simulink model "sfSelfBroadcastError"  (R2025b)
settings: Solver=VariableStepAuto  StartTime=0.0  StopTime=10.0  RelTol=1e-3
settings Model: Creator=The MathWorks, Inc.  LastModifiedBy=The MathWorks, Inc.

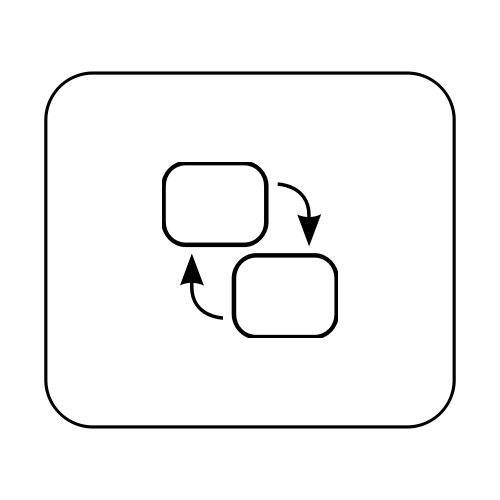
[thumbnail: Simulink's stored preview of the top-level diagram]
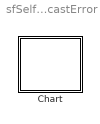
== system sfSelfBroadcastError ==
  Chart : Stateflow chart  TreatAsAtomicUnit=on

== stateflow chart sfSelfBroadcastError/Chart ==
  state A
    state B
    state C
      during:
      send(returnToSelf,A);
    (default) -> B
    B -> C
  A -> A : returnToSelf
  events: returnToSelf local FUNCTION_CALL_EVENT
